simulink model "Kirov_physics"  (R2024b)
settings: Solver=FixedStepDiscrete  StartTime=0.0  StopTime=inf  FixedStep=dt  RelTol=1e-3
undefined symbols (not defined in the file): accel_O, airspeed_bp, alpha_B, alpha_bp, alphaFull, alphaOff, b, battery_capacity_bp, battery_current_bp, battery_initial_capacity_mAh, battery_voltage_table, beta_bp, betaFull, betaOff, brake, brakes, c, channels, CLa, Clb, Clp, CLq, Clr, Cma, Cmq, Cnb, Cnp, Cnr, current_table, DiscIntNeverNeededParam, dt, ELEV_bp, elevator, f, flap, flaps, FLAPS_bp, gear, heightFadeStart, heightOff, hgt_0, Inertia_body, Inertia_load, kInduced, L_aileron, L_throttle, LAILE_bp, lat_0, lon_0, M_aile, M_body, M_elev, M_flap, M_front_gear, M_load, M_main_gear, M_prop, M_rudd, M_spoiler, minWingHeight ... (+36)
libraries: sm_lib x673, simulink x58, nesl_utility x51, simulink_extras x24, uavmavlinklib x12, instrumentlib x4, vrlib x3, aerolibfltsims x3, sharedtransform x3, eeGeneralControl x2, aerolibutil x2, AP_Connector x2
(part 1 of 6)
settings Model: DataDictionary=kirov_data.sldd  SimulationMode=accelerator  Creator=pcl  LastModifiedBy=pcl
settings DebuggingCC: InheritedTsInSrcMsg=none  ParamSuppressDoubleToSinglePrecisionLossMsg=on
settings ExplorerConfigSet: InternalSimMechanicsExplorerSettings="<ExplorerConfiguration><canonicalview>default</canonicalview><AnimationSetting><BasePlaybackSpeed>1.0</BasePlaybackSpeed><PlaybackSpeedFactor>1.0</PlaybackSpeedFactor></AnimationSetting><TilePanel><TileInfo><Tiles Columns=\"2\" Count=\"3\" Rows=\"2\"><Column Weight=\"0.5\"/><Column Weight=\"0.5\"/><Row Weight=\"0.4996\"/><Row Weight=\"0.5004\"/><Tile Height=\"2\" Width=\"1\" X=\"0\" Y=\"0\"/><Tile Height=\"1\" Width=\"1\" X=\"1\" Y=\"0\"/><Tile Height=\"1\" Width=\"1\" X=\"1\" Y=\"1\"/></Tiles></TileInfo><SceneInfo><SceneViewer><BGColor><R>0.60000002384185791</R><G>0.60000002384185791</G><B>0.60000002384185791</B></BGColor><Camera><DoPerspective>on</DoPerspective><Position><X>-41.1716710817865987</X><Y>10.006976413465603</Y><Z>20.6347061843686106</Z></Position><Center><X>-40.5943180360128224</X><Y>9.42962336769182485</Y><Z>20.0573614683873487</Z></Center><Up><X>0.408244363752572781</X><Y>-0.408244363752572892</Y><Z>0.81650050761068993</Z></Up><ViewLimDist>1</ViewLimDist><YLim>0.466307658154998583</YLim><XLim>0.394218312674211868</XLim></Camera></SceneViewer><SceneViewer><BGColor><R>0.60000002384185791</R><G>0.60000002384185791</G><B>0.60000002384185791</B></BGColor><Camera><DoPerspective>on</DoPerspective><Position><X>-11.171121143208202</X><Y>-9.99261997869194651</Y><Z>3.6314703266807622</Z></Position><Center><X>-12.1371306461597115</X><Y>-9.99265902955607466</Y><Z>3.37296377225243083</Z></Center><Up><X>-0.258506554126330057</X><Y>-1.26798323442181683e-05</Y><Z>0.966009503738422426</Z></Up><ViewLimDist>1</ViewLimDist><YLim>0.466307658154998583</YLim><XLim>0.799572735875943907</XLim></Camera></SceneViewer><SceneViewer><BGColor><R>0.60000002384185791</R><G>0.60000002384185791</G><B>0.60000002384185791</B></BGColor><Camera><DoPerspective>on</DoPerspective><Position><X>-41.1716710817865987</X><Y>10.006976413465603</Y><Z>20.6347061843686106</Z></Position><Center><X>-40.5943180360128224</X><Y>9.42962336769182485</Y><Z>20.0573614683873487</Z></Center><Up><X>0.408244363752572781</X><Y>-0.408244363752572892</Y><Z>0.81650050761068993</Z></Up><ViewLimDist>1</ViewLimDist><YLim>0.466307658154998583</YLim><XLim>0.797320418310096146</XLim></Camera></SceneViewer></SceneInfo></TilePanel><MechEditorPanel><Cameras><Camera><Id>Camera1</Id><Value><Name>LocalCam</Name><NativeCamera><PositionTrackingFeature>Dynamics.LocalFrame.R</PositionTrackingFeature><CenterTrackingFeature>Dynamics.LocalFrame.R</CenterTrackingFeature><UpVectorTrackingFeature>Dynamics.LocalFrame.R</UpVectorTrackingFeature><CenterTrackingOrigin>off</CenterTrackingOrigin><CenterTrackingDirection>+X</CenterTrackingDirection><UpVectorTrackingDirection>-Z</UpVectorTrackingDirection></NativeCamera></Value></Camera><Camera><Id>Camera2</Id><Value><Name>FollowCam</Name><NativeCamera><PositionTrackingFeature>Dynamics.FollowFrame.R</PositionTrackingFeature><CenterTrackingFeature>Dynamics.FollowFrame.R</CenterTrackingFeature><UpVectorTrackingFeature>Dynamics.FollowFrame.R</UpVectorTrackingFeature><CenterTrackingOrigin>off</CenterTrackingOrigin><CenterTrackingDirection>+X</CenterTrackingDirection><UpVectorTrackingDirection>-Z</UpVectorTrackingDirection></NativeCamera></Value></Camera><Camera><Id>Camera3</Id><Value><Name>TrackCam</Name><NativeCamera><PositionTrackingFeature>Dynamics.TrackFrame.R</PositionTrackingFeature><CenterTrackingFeature>Dynamics.TrackFrame.R</CenterTrackingFeature><UpVectorTrackingFeature>Dynamics.TrackFrame.R</UpVectorTrackingFeature><CenterTrackingOrigin>off</CenterTrackingOrigin><CenterTrackingDirection>+X</CenterTrackingDirection><UpVectorTrackingDirection>-Z</UpVectorTrackingDirection></NativeCamera></Value></Camera></Cameras><GfxPanelCameraMap><MapElement CameraMLId=\"Camera3\" GfxPanelIndex=\"0\"/><MapElement CameraMLId=\"Camera2\" GfxPanelIndex=\"1\"/><MapElement CameraMLId=\"Camera3\" GfxPanelIndex=\"2\"/></GfxPanelCameraMap><VideoCreator><PlaybackSpeedRatio>1.0</PlaybackSpeedRatio><FrameRate>30</FrameRate><VideoFormat>Motion JPEG AVI</VideoFormat><FrameSize>auto</FrameSize></VideoCreator></MechEditorPanel></ExplorerConfiguration>"

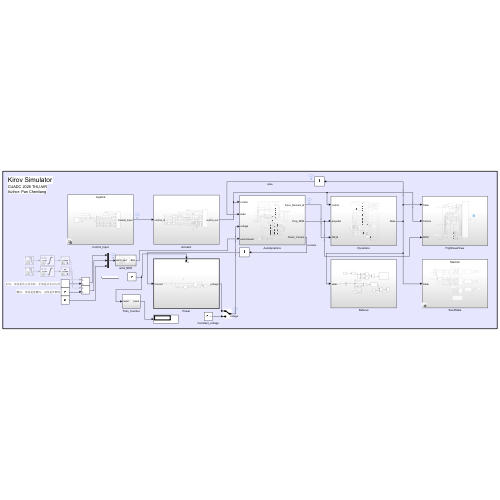
[thumbnail: Simulink's stored preview of the top-level diagram]
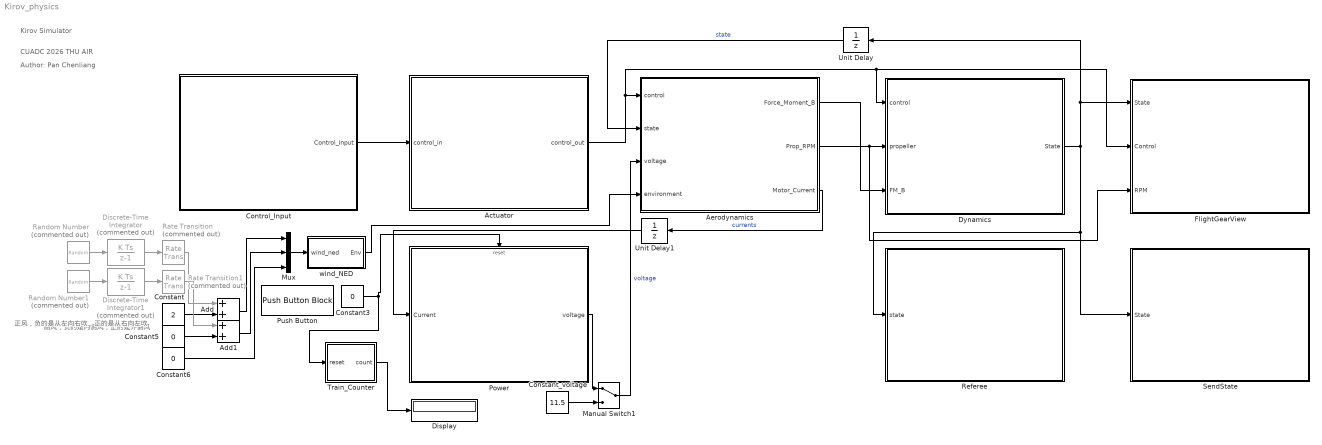
== system Kirov_physics ==
  note: CUADC 2026 THU AIR
  note: Kirov Simulator
  note: 侧风，负的是内侧风，正的是外侧风
  note: 正风，负的是从左向右吹，正的是从右向左吹
  note: Author: Pan Chenliang
  Actuator : Subsystem
  Add : Sum
  Add1 : Sum
  Aerodynamics : Subsystem
  Constant : Constant  Value=2
  Constant3 : Constant  Value=0  OutDataTypeStr=double
  Constant5 : Constant  Value=0
  Constant6 : Constant  Value=0
  Constant_voltage : Constant  Value=11.5  OutDataTypeStr=double
  Control_Input : Subsystem  Variant=on  VariantControlMode=label  VariantControl=RC  LabelModeActiveChoice=Joystick
  Discrete-Time Integrator : DiscreteIntegrator  Commented=on  SampleTime=-1  LimitOutput=on  UpperSaturationLimit=2  LowerSaturationLimit=-2  ICPrevOutput=DiscIntNeverNeededParam  ICPrevScaledInput=DiscIntNeverNeededParam
  Discrete-Time Integrator1 : DiscreteIntegrator  Commented=on  SampleTime=-1  LimitOutput=on  UpperSaturationLimit=1  LowerSaturationLimit=-1  ICPrevOutput=DiscIntNeverNeededParam  ICPrevScaledInput=DiscIntNeverNeededParam
  Display : Display
  Dynamics : Subsystem
  FlightGearView : Subsystem
  Manual Switch1 : ManualSwitch
  Mux : Mux  Inputs=3
  Power : Subsystem  TreatAsAtomicUnit=on
  Push Button : PushButtonBlock  ButtonText=Reset Battery  OffValue=0.000000
  Random Number : RandomNumber  Commented=on  Variance=2  Seed=42  SampleTime=0.05
  Random Number1 : RandomNumber  Commented=on  Seed=114514  SampleTime=0.1
  Rate Transition : RateTransition  Commented=on
  Rate Transition1 : RateTransition  Commented=on
  Referee : Subsystem
  SendState : Subsystem  Variant=on  VariantControlMode=label  LabelModeActiveChoice=Mavlink  AllowFlexibleInterface=off
  Train_Counter : Subsystem
  Unit Delay : UnitDelay  InitialCondition=struct('q',[1,0,0,0],'velocity_O',[0,0,0])  SampleTime=-1  HasFrameUpgradeWarning=on
  Unit Delay1 : UnitDelay  SampleTime=-1  HasFrameUpgradeWarning=on
  wind_NED : Subsystem
  wires:
  wind_NED/1(Env) -> Aerodynamics/4(environment)
  Mux/1 -> wind_NED/1(wind_ned)
  Unit Delay/1 -> Aerodynamics/2(state)  "state"
  Actuator/1(control_out) -> Aerodynamics/1(control), Dynamics/1(control), FlightGearView/2(Control)
  Aerodynamics/2(Prop_RPM) -> FlightGearView/3(RPM), Dynamics/2(propeller)
  Control_Input/1(Control_Input) -> Actuator/1(control_in)
  Manual Switch1/1 -> Aerodynamics/3(voltage)  "voltage"
  Aerodynamics/3(Motor_Current) -> Unit Delay1/1  "currents"
  Unit Delay1/1 -> Power/1(Current)
  Aerodynamics/1(Force_Moment_B) -> Dynamics/3(FM_B)
  Constant3/1 -> Power/Reset, Train_Counter/1(reset)
  Power/1(voltage) -> Manual Switch1/1
  Constant_voltage/1 -> Manual Switch1/2
  Constant/1 -> Add/2
  Constant5/1 -> Add1/2
  Constant6/1 -> Mux/3
  Add/1 -> Mux/1
  Add1/1 -> Mux/2
  Random Number1/1 -> Discrete-Time Integrator1/1
  Random Number/1 -> Discrete-Time Integrator/1
  Discrete-Time Integrator/1 -> Rate Transition/1
  Discrete-Time Integrator1/1 -> Rate Transition1/1
  Train_Counter/1(count) -> Display/1
  Rate Transition/1 -> Add/1
  Rate Transition1/1 -> Add1/1
  Dynamics/1(State) -> Referee/1(state), SendState/1(State), Unit Delay/1, FlightGearView/1(State)

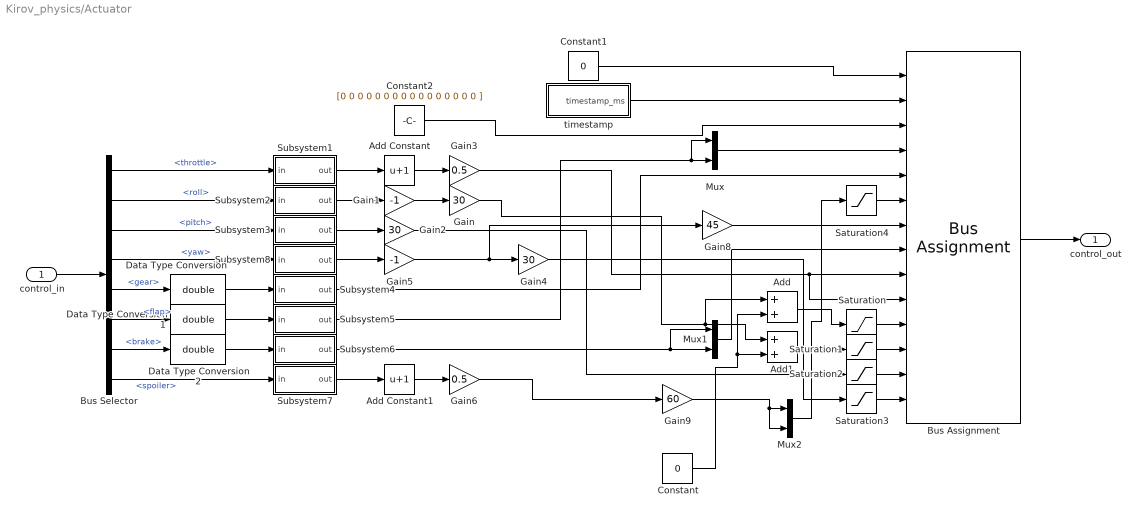
== system Kirov_physics/Actuator ==
  control_in : Inport
  Add : Sum
  Add Constant : Bias  Bias=1  SaturateOnIntegerOverflow=off
  Add Constant1 : Bias  Bias=1  SaturateOnIntegerOverflow=off
  Add1 : Sum
  Bus Assignment : BusAssignment  AssignedSignals=timestamp,channels,flaps,gear,spoilers,steer,brakes,L_throttle,R_throttle,L_aileron,R_aileron,elevator,rudder
  Bus Selector : BusSelector  OutputSignals=throttle,roll,pitch,yaw,gear,flap,brake,spoiler
  Constant : Constant  Value=0
  Constant1 : Constant  Value=0  OutDataTypeStr=Bus: Control
  Constant2 : Constant  Value=[0 0 0 0 0 0 0 0 0 0 0 0 0 0 0 0 ]  OutDataTypeStr=uint16
  Data Type Conversion : DataTypeConversion  OutDataTypeStr=double  SaturateOnIntegerOverflow=off  RndMeth=Floor
  Data Type Conversion1 : DataTypeConversion  OutDataTypeStr=double  SaturateOnIntegerOverflow=off  RndMeth=Floor
  Data Type Conversion2 : DataTypeConversion  OutDataTypeStr=double  SaturateOnIntegerOverflow=off  RndMeth=Floor
  Gain : Gain  Gain=30
  Gain1 : Gain  Gain=-1
  Gain2 : Gain  Gain=30
  Gain3 : Gain  Gain=0.5
  Gain4 : Gain  Gain=30
  Gain5 : Gain  Gain=-1
  Gain6 : Gain  Gain=0.5
  Gain8 : Gain  Gain=45
  Gain9 : Gain  Gain=60
  Mux : Mux  Inputs=2
  Mux1 : Mux  Inputs=2
  Mux2 : Mux  Inputs=2
  Saturation{,1..3} (4 alike) : Saturate  UpperLimit=30  LowerLimit=-30
  Saturation4 : Saturate  UpperLimit=60  LowerLimit=0
  Subsystem1 : Subsystem  mask{rate_limit_per_s=10, delay_s=0.1}
      mask prompts: rate_limit_per_s "rate_limit 1/s"; delay_s "delay s"
      mask DialogControl ParameterGroupVar Prompt: 参数
      mask Display: disp('Servo');
  Subsystem2 : Subsystem  mask{rate_limit_per_s=15, delay_s=0.05}
      mask prompts: rate_limit_per_s "rate_limit 1/s"; delay_s "delay s"
      mask DialogControl ParameterGroupVar Prompt: 参数
      mask Display: disp('Servo');
  Subsystem3 : Subsystem  mask{rate_limit_per_s=15, delay_s=0.05}
      mask prompts: rate_limit_per_s "rate_limit 1/s"; delay_s "delay s"
      mask DialogControl ParameterGroupVar Prompt: 参数
      mask Display: disp('Servo');
  Subsystem4 : Subsystem  mask{rate_limit_per_s=0.5, delay_s=0.2}
      mask prompts: rate_limit_per_s "rate_limit 1/s"; delay_s "delay s"
      mask DialogControl ParameterGroupVar Prompt: 参数
      mask Display: disp('Servo');
  Subsystem5 : Subsystem  mask{rate_limit_per_s=0.5, delay_s=0.2}
      mask prompts: rate_limit_per_s "rate_limit 1/s"; delay_s "delay s"
      mask DialogControl ParameterGroupVar Prompt: 参数
      mask Display: disp('Servo');
  Subsystem6 : Subsystem  mask{rate_limit_per_s=4, delay_s=0.2}
      mask prompts: rate_limit_per_s "rate_limit 1/s"; delay_s "delay s"
      mask DialogControl ParameterGroupVar Prompt: 参数
      mask Display: disp('Servo');
  Subsystem7 : Subsystem  mask{rate_limit_per_s=4, delay_s=0.1}
      mask prompts: rate_limit_per_s "rate_limit 1/s"; delay_s "delay s"
      mask DialogControl ParameterGroupVar Prompt: 参数
      mask Display: disp('Servo');
  Subsystem8 : Subsystem  mask{rate_limit_per_s=15, delay_s=0.05}
      mask prompts: rate_limit_per_s "rate_limit 1/s"; delay_s "delay s"
      mask DialogControl ParameterGroupVar Prompt: 参数
      mask Display: disp('Servo');
  timestamp : Subsystem  mask{sample_time=1000*dt}
      mask prompts: sample_time "sample time (ms)"
  control_out : Outport
  wires:
  Gain3/1 -> Bus Assignment/9, Bus Assignment/10
  Constant2/1 -> Bus Assignment/3
  Mux1/1 -> Bus Assignment/8
  timestamp/1(timestamp_ms) -> Bus Assignment/2
  Gain/1 -> Add1/1, Add/1
  Constant1/1 -> Bus Assignment/1
  Subsystem5/1(out) -> Mux/2, Mux/1
  Data Type Conversion2/1 -> Subsystem6/1(in)
  Add Constant/1 -> Gain3/1
  Mux/1 -> Bus Assignment/4
  Gain2/1 -> Saturation2/1
  Gain4/1 -> Saturation3/1
  Bus Selector/1 -> Subsystem1/1(in)  "<throttle>"
  Gain1/1 -> Gain/1
  Subsystem4/1(out) -> Bus Assignment/5
  Data Type Conversion1/1 -> Subsystem5/1(in)
  Bus Assignment/1 -> control_out/1
  Gain8/1 -> Bus Assignment/7
  Gain5/1 -> Gain8/1, Gain4/1
  Saturation/1 -> Bus Assignment/11
  Saturation1/1 -> Bus Assignment/12
  Saturation2/1 -> Bus Assignment/13
  Saturation3/1 -> Bus Assignment/14
  Add/1 -> Saturation/1
  Subsystem6/1(out) -> Mux1/2, Mux1/1
  Add1/1 -> Saturation1/1
  Gain6/1 -> Gain9/1
  Mux2/1 -> Saturation4/1
  Saturation4/1 -> Bus Assignment/6
  Gain9/1 -> Mux2/2, Mux2/1
  control_in/1 -> Bus Selector/1
  Bus Selector/2 -> Subsystem2/1(in)  "<roll>"
  Bus Selector/3 -> Subsystem3/1(in)  "<pitch>"
  Bus Selector/4 -> Subsystem8/1(in)  "<yaw>"
  Bus Selector/5 -> Data Type Conversion/1  "<gear>"
  Data Type Conversion/1 -> Subsystem4/1(in)
  Bus Selector/6 -> Data Type Conversion1/1  "<flap>"
  Bus Selector/7 -> Data Type Conversion2/1  "<brake>"
  Bus Selector/8 -> Subsystem7/1(in)  "<spoiler>"
  Subsystem1/1(out) -> Add Constant/1
  Subsystem2/1(out) -> Gain1/1
  Subsystem3/1(out) -> Gain2/1
  Subsystem8/1(out) -> Gain5/1
  Add Constant1/1 -> Gain6/1
  Subsystem7/1(out) -> Add Constant1/1
  Constant/1 -> Add1/2, Add/2

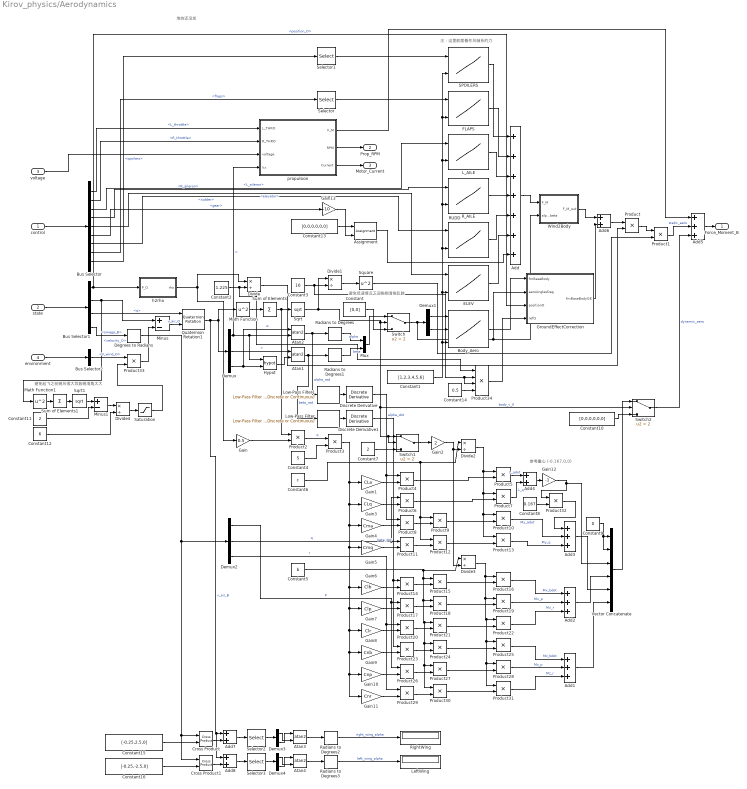
== system Kirov_physics/Aerodynamics ==
  note: 避免起飞之前侧风很大导致侧滑角太大
  note: 注：这里舵面看作风轴系的力
  note: 地效还没加
  note: 参考重心 (-0.167,0,0)
  note: 避免低速情况下迎角侧滑角乱跳
  control : Inport  OutDataTypeStr=Bus: Control  LockScale=on
  state : Inport  Port=2  OutDataTypeStr=Bus: State  LockScale=on
  voltage : Inport  Port=3
  environment : Inport  Port=4  OutDataTypeStr=Bus: Environment  LockScale=on
  Add : Sum  Inputs=+++++++
  Add{1..3,5} (4 alike) : Sum  Inputs=+++
  Add{4,6..8} (4 alike) : Sum
  Assignment : Assignment  DiagnosticForDimensions=Warning  IndexOptions=Index vector (dialog)  Indices=1  OutputSizes=1
  Atan{1..4} (4 alike) : Trigonometry  Operator=atan2
  Body_Aero : Lookup_n-D  NumberOfTableDimensions=3  BreakpointsForDimension1=alpha_bp  BreakpointsForDimension2=beta_bp  BreakpointsForDimension3=[1,2,3,4,5,6]  BeginIndexSearchUsingPreviousIndexResult=on  Table=T  InterpMethod=Linear Lagrange  ExtrapMethod=Clip  DiagnosticForOutOfRangeInput=Warning  UseLastTableValue=on  InternalRulePriority=Speed  RndMeth=Simplest
      settings: InputPortMap=u0,u1,u2
  Bus Selector : BusSelector  OutputSignals=L_throttle,R_throttle,L_aileron,R_aileron,elevator,gear,rudder,flaps,spoilers
  Bus Selector1 : BusSelector  OutputSignals=position_O,velocity_O,q,omega_B
  Bus Selector2 : BusSelector  OutputSignals=V_wind_O
  Constant : Constant  Value=[0,0]
  Constant1 : Constant  Value=[1,2,3,4,5,6]
  Constant10 : Constant  Value=[0,0,0,0,0,0]
  Constant11 : Constant  Value=2
  Constant12 : Constant  Value=6
  Constant13 : Constant  Value=[0,0,0,0,0,0]
  Constant14 : Constant  Value=0.5
  Constant15 : Constant  Value=[-0.25,2.5,0]
  Constant16 : Constant  Value=[-0.25,-2.5,0]
  Constant2 : Constant  Value=1.225
  Constant3 : Constant  Value=16
  Constant4 : Constant  Value=S
  Constant5 : Constant  Value=b
  Constant6 : Constant  Value=c
  Constant7 : Constant  Value=2
  Constant8 : Constant  Value=0.167
  Constant9 : Constant  Value=0
  Cross Product : vrlib/Utilities/Cross Product
  Cross Product1 : vrlib/Utilities/Cross Product
  Degrees to Radians : simulink_extras/Transformations/Degrees to Radians
  Demux : Demux  Outputs=3
  Demux1 : Demux  Outputs=2
  Demux2 : Demux  Outputs=3
  Demux3 : Demux  Outputs=2
  Demux4 : Demux  Outputs=2
  Discrete Derivative : simulink/Discrete/Discrete Derivative  gainval=1.0  ICPrevScaledInput=0.0  OutMin=[]  OutMax=[]  OutDataType=fixdt(1, 16)  OutScaling=2^-10  DoSatur=off
  Discrete Derivative1 : simulink/Discrete/Discrete Derivative  gainval=1.0  ICPrevScaledInput=0.0  OutMin=[]  OutMax=[]  OutDataType=fixdt(1, 16)  OutScaling=2^-10  DoSatur=off
  Divide{,1..4} (5 alike) : Product  Inputs=*/
  ELEV : Lookup_n-D  BreakpointsForDimension1=ELEV_bp  BreakpointsForDimension2=[1,2,3,4,5,6]  BeginIndexSearchUsingPreviousIndexResult=on  Table=T_ELEV  InterpMethod=Linear Lagrange  ExtrapMethod=Clip  DiagnosticForOutOfRangeInput=Error  InternalRulePriority=Speed  RndMeth=Simplest
      settings: InputPortMap=u0,u1
  FLAPS : Lookup_n-D  BreakpointsForDimension1=FLAPS_bp  BreakpointsForDimension2=[1,2,3,4,5,6]  BeginIndexSearchUsingPreviousIndexResult=on  Table=T_FLAPS  InterpMethod=Linear Lagrange  ExtrapMethod=Clip  DiagnosticForOutOfRangeInput=Error  InternalRulePriority=Speed  RndMeth=Simplest
      settings: InputPortMap=u0,u1
  Gain : Gain  Gain=0.5
  Gain1 : Gain  Gain=CLa
  Gain10 : Gain  Gain=Cnp
  Gain11 : Gain  Gain=Cnr
  Gain12 : Gain  Gain=-1
  Gain13 : Gain  Gain=-10
  Gain2 : Gain  Gain=2
  Gain3 : Gain  Gain=CLq
  Gain4 : Gain  Gain=Cma
  Gain5 : Gain  Gain=Cmq
  Gain6 : Gain  Gain=Clb
  Gain7 : Gain  Gain=Clp
  Gain8 : Gain  Gain=Clr
  Gain9 : Gain  Gain=Cnb
  GroundEffectCorrection : Subsystem
  Hypot : Math  Operator=hypot
  L_AILE : Lookup_n-D  BreakpointsForDimension1=LAILE_bp  BreakpointsForDimension2=[1,2,3,4,5,6]  BeginIndexSearchUsingPreviousIndexResult=on  Table=T_LAILE  InterpMethod=Linear Lagrange  ExtrapMethod=Clip  DiagnosticForOutOfRangeInput=Error  InternalRulePriority=Speed  RndMeth=Simplest
      settings: InputPortMap=u0,u1
  LeftWing : Display
  Low-Pass Filter : eeGeneralControl/Low-Pass Filter (Discrete or Continuous)  K=1  T=0.1  B=inf  A=-inf  init_option=Inherited from block input  x0=0  Ts=-1
  Low-Pass Filter1 : eeGeneralControl/Low-Pass Filter (Discrete or Continuous)  K=1  T=0.1  B=inf  A=-inf  init_option=Inherited from block input  x0=0  Ts=-1
  Math Function : Math  Operator=square
  Math Function1 : Math  Operator=square
  Minus : Sum  Inputs=+-
  Minus1 : Sum  Inputs=+-
  Mux : Mux  Inputs=2
  Product{,1..33} (34 alike) : Product
  Product34 : Product  Inputs=4
  Quaternion Rotation1 : aerolibutil/Quaternion Rotation
  RUDD : Lookup_n-D  BreakpointsForDimension1=RUDD_bp  BreakpointsForDimension2=[1,2,3,4,5,6]  BeginIndexSearchUsingPreviousIndexResult=on  Table=T_RUDD  InterpMethod=Linear Lagrange  ExtrapMethod=Clip  DiagnosticForOutOfRangeInput=Error  InternalRulePriority=Speed  RndMeth=Simplest
      settings: InputPortMap=u0,u1
  R_AILE : Lookup_n-D  BreakpointsForDimension1=RAILE_bp  BreakpointsForDimension2=[1,2,3,4,5,6]  BeginIndexSearchUsingPreviousIndexResult=on  Table=T_RAILE  InterpMethod=Linear Lagrange  ExtrapMethod=Clip  DiagnosticForOutOfRangeInput=Error  InternalRulePriority=Speed  RndMeth=Simplest
      settings: InputPortMap=u0,u1
  Radians to Degrees{,1..3} (4 alike) : simulink_extras/Transformations/Radians to Degrees
  RightWing : Display
  SPOILERS : Lookup_n-D  BreakpointsForDimension1=SPOILERS_bp  BreakpointsForDimension2=[1,2,3,4,5,6]  BeginIndexSearchUsingPreviousIndexResult=on  Table=T_SPOILERS  InterpMethod=Linear Lagrange  ExtrapMethod=Clip  DiagnosticForOutOfRangeInput=Error  InternalRulePriority=Speed  RndMeth=Simplest
      settings: InputPortMap=u0,u1
  Saturation : Saturate  UpperLimit=1  LowerLimit=0
  Selector : Selector  InputPortWidth=2  IndexOptions=Index vector (dialog)  Indices=[1]  OutputSizes=1
  Selector1 : Selector  InputPortWidth=2  IndexOptions=Index vector (dialog)  Indices=[1]  OutputSizes=1
  Selector2 : Selector  InputPortWidth=3  IndexOptions=Index vector (dialog)  Indices=[1 3]  OutputSizes=1
  Selector3 : Selector  InputPortWidth=3  IndexOptions=Index vector (dialog)  Indices=[1 3]  OutputSizes=1
  Sqrt : Sqrt
  Sqrt1 : Sqrt
  Square : Math  Operator=square
  Sum of Elements : Sum  Inputs=+
  Sum of Elements1 : Sum  Inputs=+
  Switch : Switch  Criteria=u2 > Threshold  Threshold=2  SaturateOnIntegerOverflow=off  InputSameDT=off
  Switch1 : Switch  Criteria=u2 > Threshold  Threshold=2  SaturateOnIntegerOverflow=off  InputSameDT=off
  Switch2 : Switch  Criteria=u2 > Threshold  Threshold=2  SaturateOnIntegerOverflow=off  InputSameDT=off
  Vector Concatenate : Concatenate  NumInputs=6
  Wind2Body : Subsystem
  h2rho : Subsystem
  propulsion : Subsystem
  Force_Moment_B : Outport
  Prop_RPM : Outport  Port=2
  Motor_Current : Outport  Port=3
  wires:
  control/1 -> Bus Selector/1
  state/1 -> Bus Selector1/1
  environment/1 -> Bus Selector2/1
  h2rho/1(rho) -> Divide/1, Gain/1
  Bus Selector1/2 -> Minus/1, Math Function1/1  "<velocity_O>"
  Product33/1 -> Minus/2
  Minus/1 -> Quaternion Rotation1/2  "v_air_O"
  Demux/3 -> Atan2/1, Hypot/2  "w"
  Math Function/1 -> Sum of Elements/1
  Atan2/1 -> Low-Pass Filter1/1, Radians to Degrees/1  "alpha_rad"
  Sqrt/1 -> Switch1/2, Switch1/1, Switch2/2, Switch/2, Divide1/1  "body_v_0"
  Hypot/1 -> Atan1/2
  Demux/2 -> Atan1/1  "v"
  Sum of Elements/1 -> Product2/1, Sqrt/1
  Atan1/1 -> Low-Pass Filter/1, Radians to Degrees1/1  "beta_rad"
  Demux/1 -> Atan2/2, Hypot/1, propulsion/4(Vx)  "u"
  Quaternion Rotation1/1 -> Demux/1, Math Function/1, Add8/1, Add7/1  "v_air_B"
  Bus Selector1/3 -> Quaternion Rotation1/1  "<q>"
  Radians to Degrees/1 -> Mux/1  "alpha"
  Radians to Degrees1/1 -> Mux/2  "beta"
  Mux/1 -> Switch/1
  Constant/1 -> Switch/3
  Bus Selector/5 -> ELEV/1  "<elevator>"
  Bus Selector/3 -> L_AILE/1  "<L_aileron>"
  Bus Selector/7 -> RUDD/1  "<rudder>"
  Bus Selector/4 -> R_AILE/1  "<R_aileron>"
  Selector/1 -> FLAPS/1
  Bus Selector/8 -> Selector/1  "<flaps>"
  Bus Selector/2 -> propulsion/2(R_THRO)  "<R_throttle>"
  Bus Selector/1 -> propulsion/1(L_THRO)  "<L_throttle>"
  L_AILE/1 -> Add/3
  R_AILE/1 -> Add/4
  RUDD/1 -> Add/5
  ELEV/1 -> Add/6
  Constant2/1 -> Product34/1, Divide/2
  Divide/1 -> Product/2
  Add6/1 -> Product/1
  Product/1 -> Product1/1
  Constant3/1 -> Product34/3, Product34/2, Divide1/2
  Divide1/1 -> Square/1
  Square/1 -> Product1/2
  Product1/1 -> Add5/2  "static_aero"
  Bus Selector1/4 -> Degrees to Radians/1  "<omega_B>"
  Demux2/2 -> Product11/1, Product6/1  "q"
  Demux2/3 -> Product29/1, Product20/1  "r"
  Gain/1 -> Product2/2
  Product2/1 -> Product3/1  "q"
  Bus Selector/9 -> Selector1/1  "<spoilers>"
  Bus Selector/6 -> Gain13/1  "<gear>"
  Discrete Derivative/1 -> Product4/1, Product8/1  "alpha_dot"
  Discrete Derivative1/1 -> Product23/1, Product14/1  "beta_dot"
  Constant4/1 -> Product3/2
  Gain1/1 -> Product4/2
  Low-Pass Filter1/1 -> Discrete Derivative/1
  Low-Pass Filter/1 -> Discrete Derivative1/1
  Gain2/1 -> Divide3/2, Divide2/2
  Switch1/1 -> Gain2/1
  Constant7/1 -> Switch1/3
  Constant6/1 -> Product12/1, Product9/1, Divide2/1
  Product4/1 -> Product5/2
  Divide2/1 -> Product13/1, Product10/1, Product7/1, Product5/1
  Product5/1 -> Add4/1  "L_adot"
  Gain3/1 -> Product6/2
  Product6/1 -> Product7/2
  Product7/1 -> Add4/2  "L_q"
  Gain4/1 -> Product8/2
  Product8/1 -> Product9/2
  Product9/1 -> Product10/2
  Product10/1 -> Add3/2  "My_adot"
  Gain5/1 -> Product11/2
  Product11/1 -> Product12/2
  Product12/1 -> Product13/2
  Product13/1 -> Add3/3  "My_q"
  Gain6/1 -> Product14/2
  Product14/1 -> Product15/2
  Product15/1 -> Product16/2
  Product16/1 -> Add2/1  "Mx_bdot"
  Product18/1 -> Product19/2
  Constant5/1 -> Product30/1, Product27/1, Product24/1, Product21/1, Product18/1, Product15/1, Divide3/1
  Product17/1 -> Product18/2
  Gain7/1 -> Product17/2
  Demux2/1 -> Product26/1, Product17/1  "p"
  Product19/1 -> Add2/2  "Mx_p"
  Gain8/1 -> Product20/2
  Product20/1 -> Product21/2
  Product21/1 -> Product22/2
  Product22/1 -> Add2/3  "Mx_r"
  Product24/1 -> Product25/2
  Product23/1 -> Product24/2
  Gain9/1 -> Product23/2
  Product25/1 -> Add1/1  "Mz_bdot"
  Gain10/1 -> Product26/2
  Product26/1 -> Product27/2
  Product27/1 -> Product28/2
  Product28/1 -> Add1/2  "Mz_p"
  Product30/1 -> Product31/2
  Product29/1 -> Product30/2
  Gain11/1 -> Product29/2
  Product3/1 -> Gain10/1, Gain11/1, Gain9/1, Gain8/1, Gain7/1, Gain6/1, Gain5/1, Gain4/1, Gain3/1, Gain1/1
  Divide3/1 -> Product25/1, Product31/1, Product28/1, Product22/1, Product19/1, Product16/1
  Product31/1 -> Add1/3  "Mz_r"
  Add2/1 -> Vector Concatenate/4
  Add1/1 -> Vector Concatenate/6
  Add4/1 -> Gain12/1
  Constant8/1 -> Product32/2
  Gain12/1 -> Vector Concatenate/3, Product32/1
  Product32/1 -> Add3/1
  Add3/1 -> Vector Concatenate/5
  Constant9/1 -> Vector Concatenate/2, Vector Concatenate/1
  Switch2/1 -> Add5/3  "dynamic_aero"
  Vector Concatenate/1 -> Switch2/1
  Constant10/1 -> Switch2/3
  voltage/1 -> propulsion/3(voltage)
  propulsion/2(RPM) -> Prop_RPM/1
  propulsion/1(F_M) -> Add5/1
  FLAPS/1 -> Add/2
  Add/1 -> Wind2Body/1(F_M)
  Wind2Body/1(F_M_out) -> Add6/1
  SPOILERS/1 -> Add/1
  Selector1/1 -> SPOILERS/1
  Gain13/1 -> Assignment/2
  Bus Selector2/1 -> Product33/1  "<V_wind_O>"
  Math Function1/1 -> Sum of Elements1/1
  Sum of Elements1/1 -> Sqrt1/1
  Sqrt1/1 -> Minus1/1
  Constant11/1 -> Minus1/2
  Minus1/1 -> Divide4/1
  Constant12/1 -> Divide4/2
  Divide4/1 -> Saturation/1
  Saturation/1 -> Product33/2
  Assignment/1 -> Add/7
  Constant13/1 -> Assignment/1
  propulsion/3(Current) -> Motor_Current/1
  GroundEffectCorrection/1(fmBaseBodyGE) -> Add6/2
  Body_Aero/1 -> GroundEffectCorrection/1(fmBaseBody)
  Add5/1 -> Force_Moment_B/1
  Constant1/1 -> FLAPS/2, SPOILERS/2, L_AILE/2, R_AILE/2, RUDD/2, ELEV/2, Body_Aero/3
  Demux1/2 -> Body_Aero/2
  Demux1/1 -> Body_Aero/1
  Switch/1 -> Wind2Body/2(alpha_beta), GroundEffectCorrection/2(aeroAnglesDeg), Demux1/1
  Bus Selector1/1 -> GroundEffectCorrection/3(positionO), h2rho/1(P_O)  "<position_O>"
  Product34/1 -> GroundEffectCorrection/4(refQ)
  Constant14/1 -> Product34/4
  Degrees to Radians/1 -> Cross Product1/1, Cross Product/1, Demux2/1
  Constant15/1 -> Cross Product/2
  Constant16/1 -> Cross Product1/2
  Cross Product/1 -> Add7/2
  Cross Product1/1 -> Add8/2
  Add7/1 -> Selector2/1
  Add8/1 -> Selector3/1
  Selector2/1 -> Demux3/1
  Demux3/2 -> Atan3/1
  Demux3/1 -> Atan3/2
  Demux4/1 -> Atan4/2
  Demux4/2 -> Atan4/1
  Selector3/1 -> Demux4/1
  Atan3/1 -> Radians to Degrees2/1
  Atan4/1 -> Radians to Degrees3/1
  Radians to Degrees2/1 -> RightWing/1  "right_wing_alpha"
  Radians to Degrees3/1 -> LeftWing/1  "left_wing_alpha"

== system Kirov_physics/Control_Input ==
  Ardupilot : Subsystem  VariantControl=Ardupilot
  Joystick : Subsystem  VariantControl=Joystick
  None : Subsystem  VariantControl=None
  Control_Input : Outport
